simulink model "RL_circuit_tostudents"  (R2021b)
settings: Solver=ode1  StartTime=0.0  StopTime=0.6  FixedStep=1e-5  RelTol=1e-3
libraries: spsControlledVoltageSourceLib x1, spsCurrentMeasurementLib x1, spsSeriesRLCBranchLib x1, spsVoltageMeasurementLib x1, spspowerguiLib x1
settings Model: Creator=Guo Qihao  LastModifiedBy=szenia
settings SolverCC: AlgebraicLoopSolver=TrustRegion
settings DebuggingCC: SFMachineParentedDataDiag=warning  ArithmeticOperatorsInVariantConditions=warning
settings SFSimCC: CustomCodeUndefinedFunction=UseInterfaceOnly

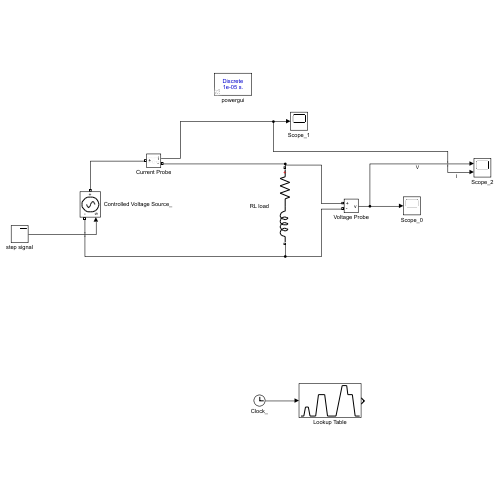
[thumbnail: Simulink's stored preview of the top-level diagram]
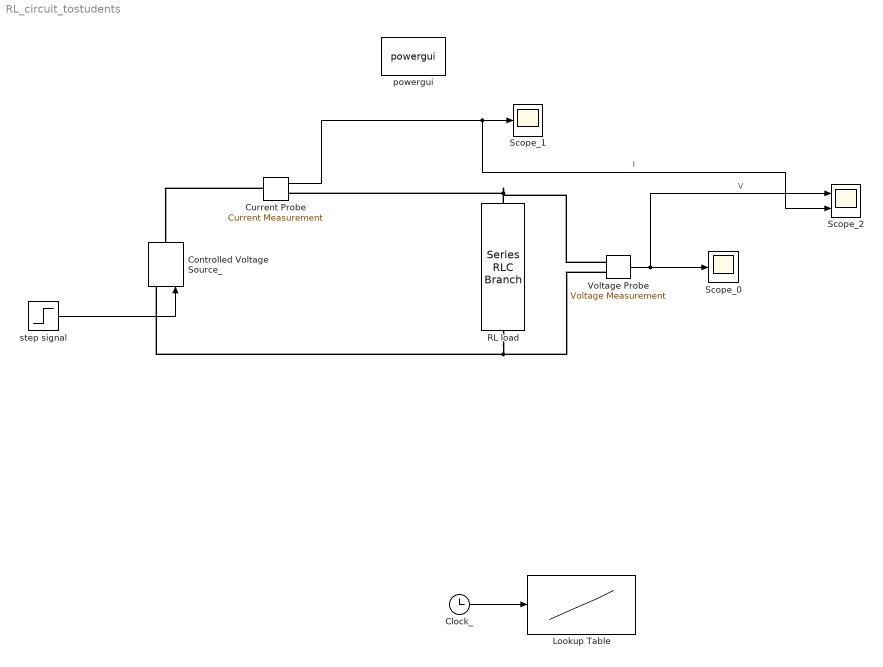
== system RL_circuit_tostudents ==
  Clock_ : Clock
  Controlled Voltage Source_ : spsControlledVoltageSourceLib/Controlled Voltage Source  Initialize=off  Source_Type=DC  Amplitude=0  Phase=0  Frequency=0  Measurements=None
  Current Probe : spsCurrentMeasurementLib/Current Measurement  PhasorSimulation=off  OutputType=Complex  PSBequivalent=0
  Lookup Table : Lookup  InputValues=[0,10,15,25,30,50,60,80,90,120,140,155,160,175,185,200]  Table=[0,0,15,15,0,0,35,35,0,0,50,50,35,35,0,0]
  RL load : spsSeriesRLCBranchLib/Series RLC Branch  LConnTagsString=__new0  RConnTagsString=__new0  BranchType=RL  Resistance=1  Inductance=1e-2  SetiL0=off  InitialCurrent=0  Capacitance=0  Setx0=off  InitialVoltage=0  Measurements=Branch current
  Scope_0 : Scope
  Scope_1 : Scope
  Scope_2 : Scope  NumInputPorts=2
  Voltage Probe : spsVoltageMeasurementLib/Voltage Measurement  PhasorSimulation=off  OutputType=Complex  PSBequivalent=0
  powergui : spspowerguiLib/powergui  Priority=1  SimulationMode=Discrete  SampleTime=1e-5  frequency=60  Iterations=50  frequencyindice=0  Pbase=100e6  ErrMax=1e-4  UnitsV=kV  UnitsW=MW  buscounter=0  FunctionMessages=off  echomessages=off  EnableUseOfTLC=off  CurrentSourceSwitches=off  DisableSnubberDevices=off  DisableRonSwitches=off  DisableVfSwitches=off  DisplayEquations=off  AutomaticDiscreteSolvers=off  SolverType=Tustin/Backward Euler (TBE)  Interpol=off  ExternalGateDelay=off  methode=off  Ts=100  x0status=zero  SPID=on  SwTol=0  HookPort=off  NonlinearTolerance=1e-4  nMaxIteration=100  ContinueOnMaxIteration=off  RestoreLinks=warning  ResistiveCurrentMeasurement=off  Frange=[0:2:500]  Ylog=off  Xlog=on  ShowGrid=off  save=off  variable=ZData  structure=0  ZoomFFT=off  StartTime=0.0  cycles=1  DisplayStyle=1  fundamental=60  FreqAxis=off  MaxFrequency=1000  frequencyindicesteady=1  RmsSteady=1  display=off
  step signal : Step  Time=0.5  Before=1  After=2  SampleTime=0
  wires:
  Current Probe/1 -> Scope_2/2, Scope_1/1  "I"
  step signal/1 -> Controlled Voltage Source_/1
  Voltage Probe/1 -> Scope_2/1, Scope_0/1  "V"
  Clock_/1 -> Lookup Table/1
  connections:
  Current Probe/LConn1 -- Controlled Voltage Source_/RConn1
  RL load/LConn1 -- Current Probe/RConn1 -- Voltage Probe/LConn1
  RL load/RConn1 -- Controlled Voltage Source_/LConn1 -- Voltage Probe/LConn2
